simulink model "gp_block_test"  (R2025b)
settings: Solver=VariableStepAuto  StartTime=0.0  StopTime=10.0  RelTol=1e-3
settings Model: Creator=HP  LastModifiedBy=HP

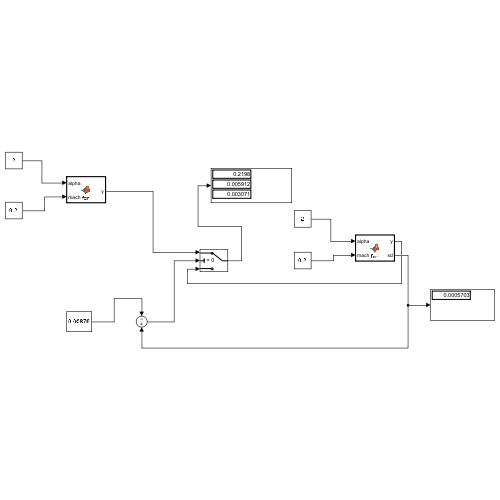
[thumbnail: Simulink's stored preview of the top-level diagram]
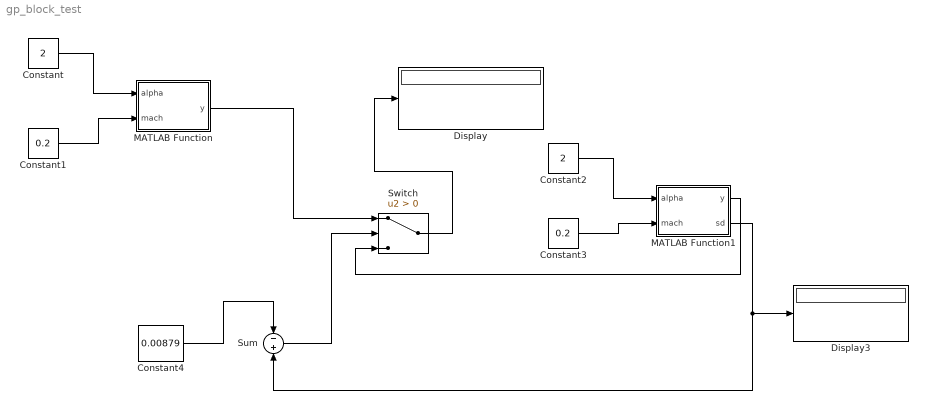
== system gp_block_test ==
  Constant : Constant  Value=2
  Constant1 : Constant  Value=0.2
  Constant2 : Constant  Value=2
  Constant3 : Constant  Value=0.2
  Constant4 : Constant  Value=0.00879
  Display : Display
  Display3 : Display
  MATLAB Function : MATLAB Function  TreatAsAtomicUnit=on
  MATLAB Function1 : MATLAB Function  TreatAsAtomicUnit=on
  Sum : Sum  Inputs=-+
  Switch : Switch  Criteria=u2 > Threshold  SaturateOnIntegerOverflow=off  InputSameDT=off
  wires:
  Constant/1 -> MATLAB Function/1(alpha)
  Constant1/1 -> MATLAB Function/2(mach)
  MATLAB Function/1(y) -> Switch/1
  Constant3/1 -> MATLAB Function1/2(mach)
  Constant2/1 -> MATLAB Function1/1(alpha)
  Constant4/1 -> Sum/1
  MATLAB Function1/2(sd) -> Display3/1, Sum/2
  Sum/1 -> Switch/2
  MATLAB Function1/1(y) -> Switch/3
  Switch/1 -> Display/1

== matlab function gp_block_test/MATLAB Function1 ==
  data: alpha input; y output; mach input; sd output
function [y, sd] = fcn(alpha, mach)
coder.extrinsic('gp_predict');
y  = zeros(1,3);
sd = 0;
[y, sd] = gp_predict(alpha, mach);
end

== matlab function gp_block_test/MATLAB Function ==
  data: alpha input; y output; mach input
function y = fcn(alpha, mach)
coder.extrinsic('lookup_predict');
y = zeros(1,3);
y = lookup_predict(alpha, mach);
end
